simulink model "Simulacion_Ideal"  (R2026a)
settings: Solver=VariableStepAuto  StopTime=2000
model workspace (MAT data in the model file):
  Tref = Simulink.Parameter
  Tref.Complexity = 'real'
  Tref.Dimensions = [0 0]
  Tref.DataType = 'auto'
values from neighbouring files (symbols this model uses):
  K = 0.1316    [ControlAnalitico.m]    (also in ModeladoLCA.m = 0.13155478989)
  Ki = 1 / (K * tau_cl)    (= 0.0506585612969)    [ControlAnalitico.m]    (also in PIDnuevo.m = 0.0016)
  Kp = tau / (K * tau_cl)    (= 8.43465045593)    [ControlAnalitico.m]    (also in PIDnuevo.m = 0.85)
  tau = 166.5    [ControlAnalitico.m]    (also in ModeladoLCA.m = 166.512148502)
settings Model: Creator=Mariano M  LastModifiedBy=Mariano M

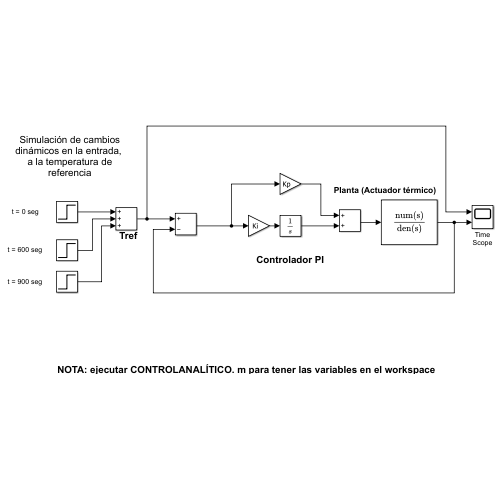
[thumbnail: Simulink's stored preview of the top-level diagram]
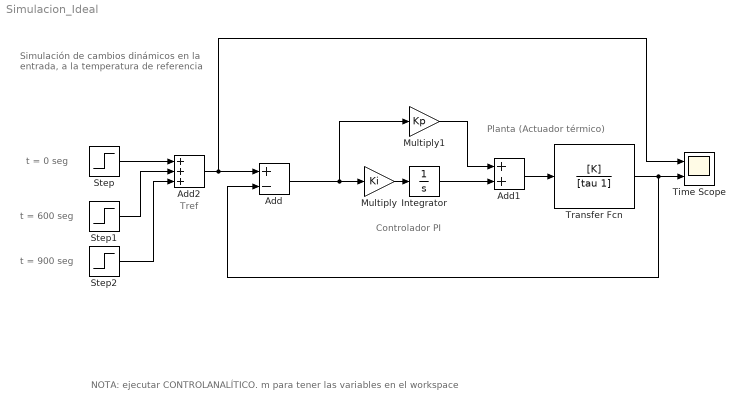
== system Simulacion_Ideal ==
  note: NOTA: ejecutar CONTROLANALÍTICO. m para tener las variables en el workspace
  note: Controlador PI
  note: t = 0 seg
  note: Tref
  note: Simulación de cambios
      | dinámicos en la entrada,
      | a la temperatura de referencia
  note: t = 600 seg
  note: t = 900 seg
  note: Planta (Actuador térmico)
  Add : Sum  Inputs=+-
  Add1 : Sum
  Add2 : Sum  Inputs=+++
  Integrator : Integrator
  Multiply : Gain  Gain=Ki
  Multiply1 : Gain  Gain=Kp
  Step : Step  Time=0  FinalValue=15  SampleTime=0
  Step1 : Step  Time=600  FinalValue=15  SampleTime=0
  Step2 : Step  Time=900  FinalValue=15  SampleTime=0
  Time Scope : Scope  NumInputPorts=2
      settings: TimeUnits=Metric (based on Time Span)  ActiveDisplayYMinimum=0  ActiveDisplayYMaximum=100  YLabel=Amplitude
  Transfer Fcn : TransferFcn  Numerator=[K]  Denominator=[tau 1]
  wires:
  Transfer Fcn/1 -> Time Scope/2, Add/2
  Add2/1 -> Time Scope/1, Add/1
  Add/1 -> Multiply1/1, Multiply/1
  Multiply/1 -> Integrator/1
  Integrator/1 -> Add1/2
  Add1/1 -> Transfer Fcn/1
  Multiply1/1 -> Add1/1
  Step/1 -> Add2/1
  Step1/1 -> Add2/2
  Step2/1 -> Add2/3
